simulink library "Multibody_Parts_Lib"  (R2025a)
settings: Solver=VariableStepAuto  StartTime=0.0  StopTime=10.0  RelTol=1e-3
undefined symbols (not defined in the file): b_gear_pd_asy, b_radius_asy, b_visc_frict_asy, bevel_angle_asy, bevel_angle_bf_asy, bevel_angle_fg_asy, f_gear_pd_asy, f_radius_asy, f_visc_frict_asy, g_radius_asy, g_visc_frict_asy, gear_ra_asy, gear_visc_frict_asy, Hand, Left, Local, pinion_pd_asy, screw_lead, worm_lead_angle_asy, worm_rad_asy, worm_visc_frict_asy, X, Y, Z
libraries: sm_lib x143, $bdroot x22, nesl_utility x16
(part 1 of 6)
Description:
  | Simscape Multibody Parts Library v4.0
  | Copyright 2018-2025 The MathWorks, Inc.
settings Model: Creator=smiller  LastModifiedBy=smiller
settings SolverCC: AlgebraicLoopSolver=TrustRegion
settings DataIOCC: ReturnWorkspaceOutputs=off
settings OptimizationCC: ReuseModelBlockBuffer=off
settings DebuggingCC: UnconnectedInputMsg=warning  UnconnectedOutputMsg=warning  UnconnectedLineMsg=warning  PregeneratedLibrarySubsystemCodeDiagnostic=none  ArithmeticOperatorsInVariantConditions=warning
settings ModelReferenceCC: EnableRefExpFcnMdlSchedulingChecks=on
settings SFSimCC: SimUseLocalCustomCode=off  CustomCodeUndefinedFunction=UseInterfaceOnly
settings RTWCC: RTWUseLocalCustomCode=off  GPUComputeCapability=3.5  DLArmComputeVersion=19.05
settings CodeAppCC: StateflowObjectComments=on

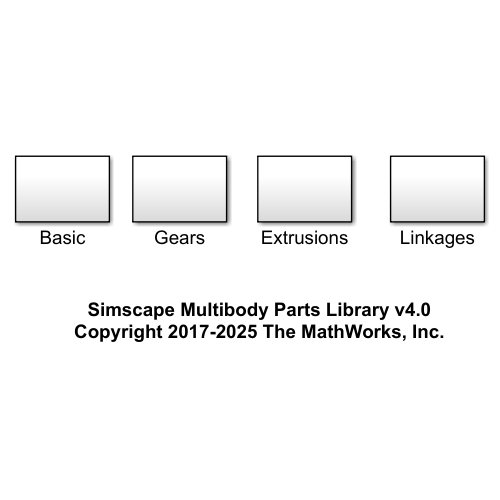
[thumbnail: Simulink's stored preview of the top-level diagram]
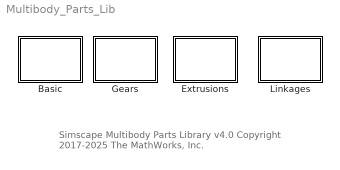
== system Multibody_Parts_Lib ==
  note: Simscape Multibody Parts Library v4.0
      | Copyright 2017-2025 The MathWorks, Inc.
  Basic : Subsystem
  Extrusions : Subsystem
  Gears : Subsystem
  Linkages : Subsystem

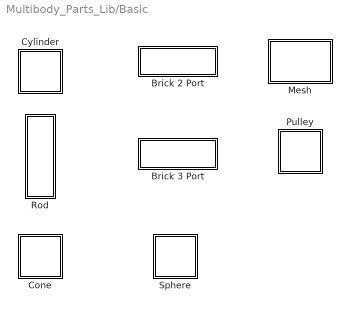
== system Multibody_Parts_Lib/Basic ==
  Brick 2 Port : Subsystem  mask(Brick with 2 Interface Frames){len_xyz=[0.1 0.2 0.3], brick_rho=7000, brick_clr=[0.6 0.6 0.6], brick_opc=1, popup_port1=+X, popup_port2=+X, port1_offset=[0 0 0]}
      mask prompts: len_xyz "Length [X Y Z] (m)"; brick_rho "Density (kg/m^3)"; brick_clr "Color [RGB]"; brick_opc "Opacity (0-1)"; popup_port1 "Port 1 Face"; popup_port2 "Port 2 Face"
      mask help: This block models a brick. The two interface ports can be configured to be at the center of any of the six faces. The orientation of the frames is the same.
      mask init:
      | f=Simulink.FindOptions('FollowLinks',1,'LookUnderMasks','all');
      | p1_h=Simulink.findBlocks(gcb,'Port','1',f);
      | p2_h=Simulink.findBlocks(gcb,'Port','2',f);
      | 
      | switch(popup_port1)
      |     case 1, port1_offset = [ len_xyz(1)/2 0 0]; port1_name = '1X';
      |     case 2, port1_offset = [-len_xyz(1)/2 0 0];  port1_name = '1-X';
      |     case 3, port1_offset = [ 0  len_xyz(2)/2 0];  port1_name = '1Y';
      |     case 4, port1_offset = [ 0 -len_xyz(2)/2 0];  port1_name = '1-Y';
      |     case 5, port1_offset = [ 0  0  len_xyz(3)/2]; port1_name = '1Z';
      |     case 6, port1_offset = [ 0  0 -len_xyz(3)/2]; port1_name = '1-Z';
      | end
      | 
      | switch(popup_port2)
      |     case 1, port2_offset = [ len_xyz(1)/2 0 0]; port2_name = 'X2';
      |     case 2, port2_offset = [-len_xyz(1)/2 0 0];  port2_name = '-X2';
      |     case 3, port2_offset = [ 0  len_xyz(2)/2 0];  port2_name = 'Y2';
      |     case 4, port2_offset = [ 0 -len_xyz(2)/2 0];  port2_name = '-Y2';
      |     case 5, port2_offset = [ 0  0  len_xyz(3)/2]; port2_name = 'Z2';
      |     case 6, port2_offset = [ 0  0 -len_xyz(3)/2]; port2_name = '-Z2';
      | end
      | 
      | set_param(p1_h,'Name',port1_name);
      | set_param(p2_h,'Name',port2_name);
      mask TypeOptions popup_port1: +X | -X | +Y | -Y | +Z | -Z
      mask TypeOptions popup_port2: +X | -X | +Y | -Y | +Z | -Z
      mask Display: image('Brick_2_Port_IMAGE.png')
  Brick 3 Port : Subsystem  mask(Brick with 3 Interface Frames){len_xyz=[0.1 0.2 0.3], brick_rho=7000, brick_clr=[0.6 0.6 0.6], brick_opc=1, popup_port1=+X, popup_port2=+X, popup_port3=+X, port1_offset=[0 0 0]}
      mask prompts: len_xyz "Length [X Y Z] (m)"; brick_rho "Density (kg/m^3)"; brick_clr "Color [RGB]"; brick_opc "Opacity (0-1)"; popup_port1 "Port 1 Face"; popup_port2 "Port 2 Face"; popup_port3 "Port 3 Face"
      mask help: This block models a brick. The three interface ports can be configured to be at the center of any of the six faces. The orientation of the frames is the same.
      mask init:
      | f=Simulink.FindOptions('FollowLinks',1,'LookUnderMasks','all');
      | p1_h=Simulink.findBlocks(gcb,'Port','1',f);
      | p2_h=Simulink.findBlocks(gcb,'Port','2',f);
      | p3_h=Simulink.findBlocks(gcb,'Port','3',f);
      | 
      | switch(popup_port1)
      |     case 1, port1_offset = [ len_xyz(1)/2 0 0]; port1_name = '1X';
      |     case 2, port1_offset = [-len_xyz(1)/2 0 0];  port1_name = '1-X';
      |     case 3, port1_offset = [ 0  len_xyz(2)/2 0];  port1_name = '1Y';
      |     case 4, port1_offset = [ 0 -len_xyz(2)/2 0];  port1_name = '1-Y';
      |     case 5, port1_offset = [ 0  0  len_xyz(3)/2]; port1_name = '1Z';
      |     case 6, port1_offset = [ 0  0 -len_xyz(3)/2]; port1_name = '1-Z';
      | end
      | 
      | switch(popup_port2)
      |     case 1, port2_offset = [ len_xyz(1)/2 0 0]; port2_name = 'X2';
      |     case 2, port2_offset = [-len_xyz(1)/2 0 0];  port2_name = '-X2';
      |     case 3, port2_offset = [ 0  len_xyz(2)/2 0];  port2_name = 'Y2';
      |     case 4, port2_offset = [ 0 -len_xyz(2)/2 0];  port2_name = '-Y2';
      |     case 5, port2_offset = [ 0  0  len_xyz(3)/2]; port2_name = 'Z2';
      |     case 6, port2_offset = [ 0  0 -len_xyz(3)/2]; port2_name = '-Z2';
      | end
      | 
      | switch(popup_port3)
      |     case 1, port3_offset = [ len_xyz(1)/2 0 0]; port3_name = 'X3';
      |     case 2, port3_offset = [-len_xyz(1)/2 0 0];  port3_name = '-X3';
      |     case 3, port3_offset = [ 0  len_xyz(2)/2 0];  port3_name = 'Y3';
      |     case 4, port3_offset = [ 0 -len_xyz(2)/2 0];  port3_name = '-Y3';
      |     case 5, port3_offset = [ 0  0  len_xyz(3)/2]; port3_name = 'Z3';
      |     case 6, port3_offset = [ 0  0 -len_xyz(3)/2]; port3_name = '-Z3';
      | end
      | 
      | set_param(p1_h,'Name',port1_name);
      | set_param(p2_h,'Name',port2_name);
      | set_param(p3_h,'Name',port3_name);
      mask TypeOptions popup_port1: +X | -X | +Y | -Y | +Z | -Z
      mask TypeOptions popup_port2: +X | -X | +Y | -Y | +Z | -Z
      mask TypeOptions popup_port3: +X | -X | +Y | -Y | +Z | -Z
      mask Display: image('Brick_3_Port_IMAGE.png');
  Cone : Subsystem  mask(Conical Frustum){cone_or=37.5e-3, cone_ir=30e-3, cone_h=4e-2, cone_theta=60, cone_angle_range=[-180 180], cone_rho=7000, cone_clr=[0.0 0.4 0.6], cone_opc=1, popup_markings=Two, mark_radius_scale=[1.01 1.01], mark_angle_range=2, mark_color=[1 1 1]}
      mask prompts: cone_or "Outer Radius (m):"; cone_ir "Inner Radius (m):"; cone_h "Height (m):"; cone_theta "Angle (deg):"; cone_angle_range "Sweep Angle (min, max angle (deg))"; cone_rho "Density (kg/m^3):"; cone_clr "Color [RGB]:"; cone_opc "Opacity (0-1)"; popup_markings "Show Markings"; mark_radius_scale "Radius scale factor [rad, h] (~1)"; mark_angle_range "Sweep Angle [0-180] (deg)"; mark_color "Color [RGB]"
      mask help:
      | This block models a conical frustum.
      |
      | The port C corresponds to the frame at one end of the cone whose z-axis points along the cone axis.
      mask init:
      | frcon_xsec = Extr_Data_Frustum_Conical(cone_or, cone_theta, cone_h, cone_ir);
      | mark_xsec = Extr_Data_Frustum_Conical(cone_or*mark_radius_scale(1), cone_theta, cone_h*(1+(mark_radius_scale(2)-1)*2), cone_ir*(2-mark_radius_scale(1)));
      | 
      | mark_xsec(:,2) = mark_xsec(:,2)-cone_h*(mark_radius_scale(2)-1);
      | 
      | mark_1_opc = 0;
      | mark_2_opc = 0;
      | 
      | if(popup_markings == 2)
      |     mark_1_opc = 1;
      | elseif(popup_markings == 3)
      |     mark_1_opc = 1;
      |     mark_2_opc = 1;
      | end
      mask TypeOptions popup_markings: None | One | Two
      mask Callback popup_markings:
      | maskObj = Simulink.Mask.get(gcb);
      | mkc_h = maskObj.getDialogControl('container_markings');
      | if strcmp(get_param(gcb,'popup_markings'),'None')
      |     mkc_h.Visible = 'off';
      | else
      |     mkc_h.Visible = 'on';
      | end
      | clear maskObj mkc_h
      mask DialogControl Control2 Prompt: Plot Profile
      mask DialogControl Control2 Callback:
      | v = get_param(gcb,'MaskWSVariables');
      | getMaskValue = containers.Map({v.Name}',{v.Value}');
      | evalin('base',...
      |     sprintf('Extr_Data_Frustum_Conical(%s,%s,%s,%s,''%s'');',...
      |     num2str(getMaskValue('cone_or')),...
      |     num2str(getMaskValue('cone_theta')),...
      |     num2str(getMaskValue('cone_h')),...
      |     num2str(getMaskValue('cone_ir')),'plot'));
      mask Display: image('Cone_IMAGE.png');
  Cylinder : Subsystem  mask(Cylinder with Hole){cyl_ra=37.5e-3, cyl_th=9e-3, cyl_hr=5e-3, cyl_rho=7000, cyl_clr=[0.6 0.6 0.6], cyl_opc=1, popup_markings=Two, mark_radius_range=[0.7 0.9], mark_angle_range=60, mark_color=[1 1 1]}
      mask prompts: cyl_ra "Radius (m):"; cyl_th "Length (m):"; cyl_hr "Hole Radius (m):"; cyl_rho "Density (kg/m^3):"; cyl_clr "Color [RGB]:"; cyl_opc "Opacity (0-1):"; popup_markings "Show Markings"; mark_radius_range "Radial Range [min max] (0-1)"; mark_angle_range "Sweep Angle [0-180] (deg)"; mark_color "Color [RGB]"
      mask help:
      | This block models a cylinder with a hole for the shaft.
      |
      | The port C corresponds to the frame at the center of the cylinder.
      mask init:
      | cyl_xsec = [cyl_hr -cyl_th/2;
      |              cyl_ra -cyl_th/2;
      |              cyl_ra cyl_th/2;
      |              cyl_hr cyl_th/2];
      | mark_xsec =  [
      |     cyl_ra*max(mark_radius_range) cyl_th/1.9; 
      |     cyl_ra*min(mark_radius_range) cyl_th/1.9; 
      |     cyl_ra*min(mark_radius_range) -cyl_th/1.9; 
      |     cyl_ra*max(mark_radius_range) -cyl_th/1.9];
      | 
      | mark_1_opc = 0;
      | mark_2_opc = 0;
      | 
      | if(popup_markings == 2)
      |     mark_1_opc = 1;
      | elseif(popup_markings == 3)
      |     mark_1_opc = 1;
      |     mark_2_opc = 1;
      | end
      mask TypeOptions popup_markings: None | One | Two
      mask Callback popup_markings:
      | maskObj = Simulink.Mask.get(gcb);
      | mkc_h = maskObj.getDialogControl('container_markings');
      | if strcmp(get_param(gcb,'popup_markings'),'None')
      |     mkc_h.Visible = 'off';
      | else
      |     mkc_h.Visible = 'on';
      | end
      | clear maskObj mkc_h
      mask Display: image('Cylinder_IMAGE.png');
  Mesh : Subsystem  mask(Rectangular Mesh){mesh_lenx=0.6, mesh_leny=0.4, mesh_hx=0.18, mesh_hy=0.18, mesh_numhx=3, mesh_numhy=2, mesh_thickness=0.02, mesh_rho=7000, mesh_color=[0 0.4 0.6], mesh_opc=1}
      mask prompts: mesh_thickness "Thickness (m)"; mesh_rho "Density (kg/m^3)"; mesh_color "Color [RGB]"; mesh_opc "Opacity (0-1)"
      mask help: Rectangular mesh. Define outer dimensions, dimensions of holes, and thickness. R port is at the CG. Thickness defines the distance of the F frame from the B frame along the z-axis.
      mask init:
      | mesh_xsec = Extr_Data_Mesh(mesh_lenx, mesh_leny, mesh_numhx, mesh_numhy, mesh_hx, mesh_hy);
      mask DialogControl Control12 Prompt: Plot Profile
      mask DialogControl Control12 Callback:
      | v = get_param(gcb,'MaskWSVariables');
      | getMaskValue = containers.Map({v.Name}',{v.Value}');
      | evalin('base',...
      |     sprintf('Extr_Data_Mesh(%s,%s,%s,%s,%s,%s,''%s'');',...
      |     num2str(getMaskValue('mesh_lenx')),...
      |     num2str(getMaskValue('mesh_leny')),...
      |     num2str(getMaskValue('mesh_numhx')),...
      |     num2str(getMaskValue('mesh_numhy')),...
      |     num2str(getMaskValue('mesh_hx')),...
      |     num2str(getMaskValue('mesh_hy')),'plot'));
      mask DialogControl Control7 Prompt: X
      mask DialogControl Control8 Prompt: Y
      mask DialogControl Control9 Prompt: Mesh Length (m)
      mask DialogControl Control11 Prompt: Hole Length (m)
      mask DialogControl Control10 Prompt: Number of Holes
      mask Display: image('Mesh_IMAGE.png');
  Pulley : Subsystem  mask(Pulley with Hole){pulley_rad=0.02, pulley_d_grv=0.005, pulley_a_grv=45, pulley_th=0.01, pulley_radh=0.005, pulley_rho=7000, pulley_clr=[0.6 0.6 0.6], pulley_opc=1, pulley_zori=No, popup_markings=Two, mark_radius_range=[0.7 0.9], mark_angle_range=60, mark_color=[1 1 1]}
      mask prompts: pulley_rad "Radius for Cable (m):"; pulley_d_grv "Groove Depth (m):"; pulley_a_grv "Groove Angle (deg):"; pulley_th "Pulley Thickness (m):"; pulley_radh "Hole Radius (m):"; pulley_rho "Density (kg/m^3):"; pulley_clr "Color [RGB]:"; pulley_opc "Opacity (0-1)"; pulley_zori "Flip Z Axis"; popup_markings "Show Markings"; mark_radius_range "Radial Range [min max] (0-1)"; mark_angle_range "Sweep Angle [0-180] (deg)"; mark_color "Color [RGB]"
      mask help:
      | This block models a pulley with a groove for a cable and a hole for the shaft.
      |
      | The port C corresponds to the frame at the center of the pulley.
      mask init:
      | pulley_xsec = Extr_Data_Pulley(...
      |     pulley_rad, pulley_d_grv, pulley_radh,...
      |     pulley_a_grv, pulley_th);
      | 
      | mark_xsec =  [
      |     pulley_rad*max(mark_radius_range) pulley_th/1.9; 
      |     pulley_rad*min(mark_radius_range) pulley_th/1.9; 
      |     pulley_rad*min(mark_radius_range) -pulley_th/1.9; 
      |     pulley_rad*max(mark_radius_range) -pulley_th/1.9];
      | 
      | mark_1_opc = 0;
      | mark_2_opc = 0;
      | 
      | if(pulley_zori == 1)
      |  set_param([gcb '/Transform Swap Z'],'RotationMethod','None'),
      | elseif(pulley_zori == 2)
      |  set_param([gcb '/Transform Swap Z'],'RotationMethod','StandardAxis','RotationStandardAxis','+X'),
      | elseif(pulley_zori == 3)
      |  set_param([gcb '/Transform Swap Z'],'RotationMethod','StandardAxis','RotationStandardAxis','+Y'),
      | end    
      | 
      | if(popup_markings == 2)
      |     mark_1_opc = 1;
      | elseif(popup_markings == 3)
      |     mark_1_opc = 1;
      |     mark_2_opc = 1;
      | end
      mask TypeOptions pulley_zori: No | Yes, about X | Yes, about Y
      mask TypeOptions popup_markings: None | One | Two
      mask Callback popup_markings:
      | maskObj = Simulink.Mask.get(gcb);
      | mkc_h = maskObj.getDialogControl('container_markings');
      | if strcmp(get_param(gcb,'popup_markings'),'None')
      |     mkc_h.Visible = 'off';
      | else
      |     mkc_h.Visible = 'on';
      | end
      | clear maskObj mkc_h
      mask DialogControl Control2 Prompt: Plot Profile
      mask DialogControl Control2 Callback:
      | v = get_param(gcb,'MaskWSVariables');
      | getMaskValue = containers.Map({v.Name}',{v.Value}');
      | evalin('base',...
      |     sprintf('Extr_Data_Pulley(%s,%s,%s,%s,%s,''%s'');',...
      |     num2str(getMaskValue('pulley_rad')),...
      |     num2str(getMaskValue('pulley_d_grv')),...
      |     num2str(getMaskValue('pulley_radh')),...
      |     num2str(getMaskValue('pulley_a_grv')),...
      |     num2str(getMaskValue('pulley_th')),'plot'));
      mask Display: image('Pulley_IMAGE.png');
  Rod : Subsystem  mask(Rod){rod_rad=0.005, rod_len=0.0125, rod_rho=7000, rod_color=[0.5 0.5 0.5], rod_opc=1, popup_zori=Local +Z, popup_markings=None, mark_radius_range=[0.5 1.01], mark_length_range=1.005, mark_angle_range=30, mark_color=[1 1 1]}
      mask prompts: rod_rad "Radius (m)"; rod_len "Length (m)"; rod_rho "Density (kg/m^3)"; rod_color "Color [RGB]"; rod_opc "Opacity (0-1)"; popup_zori "Relative Position (B to F)"; popup_markings "Show Markings"; mark_radius_range "Radial Range [min max] (0-1.1)"; mark_length_range "Length Range (0-1.1)"; mark_angle_range "Sweep Angle [0-180] (deg)"; mark_color "Color [RGB]"
      mask help:
      | This block models a rod.
      |
      | The two interface ports corresponds to the frames at either end of the rod which are along the z-axis.
      mask init:
      | mark_xsec =  [
      |     rod_rad*max(mark_radius_range) rod_len*mark_length_range/2; 
      |     rod_rad*min(mark_radius_range) rod_len*mark_length_range/2; 
      |     rod_rad*min(mark_radius_range) -rod_len*mark_length_range/2; 
      |     rod_rad*max(mark_radius_range) -rod_len*mark_length_range/2];
      | 
      | mark_1_opc = 0;
      | mark_2_opc = 0;
      | 
      | if(popup_markings == 2)
      |     mark_1_opc = 1;
      | elseif(popup_markings == 3)
      |     mark_1_opc = 1;
      |     mark_2_opc = 1;
      | end
      | 
      | if(popup_zori == 2)
      |     z_ori = -1;
      | else
      |     z_ori = 1;
      | end
      mask TypeOptions popup_zori: Local +Z | Local -Z
      mask TypeOptions popup_markings: None | One | Two
      mask Callback popup_markings:
      | maskObj = Simulink.Mask.get(gcb);
      | mkc_h = maskObj.getDialogControl('container_markings');
      | if strcmp(get_param(gcb,'popup_markings'),'None')
      |     mkc_h.Visible = 'off';
      | else
      |     mkc_h.Visible = 'on';
      | end
      | clear maskObj mkc_h
      mask Display:
      | if(popup_zori == 2)
      |     image('Rod_nZ_IMAGE.png')
      | else
      |     image('Rod_pZ_IMAGE.png')
      | end
  Sphere : Subsystem  Tag=CustomStyle  mask(Sphere){sph_radius=0.01, sph_density=1000, sph_color=[0 0.4 0.6], sph_opacity=1, mark_type=Arcs about axes, arc_width=[40 50], arc_angle=60, ring_width=5, ring_irad=0.95, mark_color_popup=Axes, mark_color=[0.2 0.2 0.2], mark_color_x=[1 0 0];, mark_color_y=[0 1 0];, mark_color_z=[0 0 1];, mark_opacity_x=1, mark_opacity_y=1, mark_opacity_z=1, mark_opacity=1, ring_opacity=0, arc_opacity=0, arc_extr_data=0}
      mask prompts: sph_radius "Radius (m)"; sph_density "Density (kg/m^3)"; sph_color "Color [RGB]"; sph_opacity "Opacity"; mark_type "Marking Type"; arc_width "Arc width (start, end) (deg)"; arc_angle "Sweep angle (deg)"; ring_width "Ring Width (deg)"; ring_irad "Ring Inner Radius (% sphere radius)"; mark_color_popup "Color Scheme"; mark_color "Color [RGB]"; mark_opacity_x "Opacity (0-1): X-Axis"; mark_opacity_y "Y-Axis"; mark_opacity_z "Z-Axis"; mark_opacity "Opacity"; ring_opacity "Ring Opacity"; arc_opacity "Arc Opacity"; arc_extr_data "Arc Extrusion Data (xy)"
      mask help:
      | This block models a sphere.
      |
      | The port C corresponds to the frame at the center of the sphere.
      mask init:
      | curblk = gcb;
      | 
      | if strcmp(get_param(curblk,'mark_color_popup'),'Axes')
      |     mark_color_x = [1.0 0.0 0.0];
      |     mark_color_y = [0.0 1.0 0.0];
      |     mark_color_z = [0.0 0.0 1.0];
      | else
      |     mark_color_x = mark_color;
      |     mark_color_y = mark_color;
      |     mark_color_z = mark_color;
      | end
      | 
      | arc_opacity = 0;
      | ring_opacity = 0;
      | 
      | if strcmp(get_param(curblk,'mark_type'),'Arcs about axes')
      |     arc_opacity = 1;
      | elseif strcmp(get_param(curblk,'mark_type'),'Rings on center planes')
      |     ring_opacity = 1;
      | end
      | 
      | arc_extr_data = sph_radius*1.0001*[cosd(min(arc_width):(max(arc_width)-min(arc_width))/20:max(arc_width)) cosd(-max(arc_width):(max(arc_width)-min(arc_width))/20:-min(arc_width)); sind(min(arc_width):(max(arc_width)-min(arc_width))/20:max(arc_width)) sind(-max(arc_width):(max(arc_width)-min(arc_width))/20:-min(arc_width))]';
      | clear curblk
      mask TypeOptions mark_type: None | Arcs about axes | Rings on center planes
      mask Callback mark_type:
      | maskObj = Simulink.Mask.get(gcb);
      | arw_h = maskObj.getParameter('arc_width');
      | ara_h = maskObj.getParameter('arc_angle');
      | riw_h = maskObj.getParameter('ring_width');
      | rii_h = maskObj.getParameter('ring_irad');
      | mkp_h = maskObj.getParameter('mark_color_popup');
      | mkc_h = maskObj.getParameter('mark_color');
      | opx_h = maskObj.getParameter('mark_opacity_x');
      | opy_h = maskObj.getParameter('mark_opacity_y');
      | opz_h = maskObj.getParameter('mark_opacity_z');
      |     arw_h.Visible = 'off';
      |     ara_h.Visible = 'off';
      |     riw_h.Visible = 'off';
      |     rii_h.Visible = 'off';
      |     mkp_h.Visible = 'off';
      |     mkc_h.Visible = 'off';
      |     opx_h.Visible = 'off';
      |     opy_h.Visible = 'off';
      |     opz_h.Visible = 'off';
      | if strcmp(get_param(gcb,'mark_type'),'Arcs about axes')
      |     arw_h.Visible = 'on';
      |     ara_h.Visible = 'on';
      |     mkp_h.Visible = 'on';
      |     mkc_h.Visible = 'on';
      |     opx_h.Visible = 'on';
      |     opy_h.Visible = 'on';
      |     opz_h.Visible = 'on';
      | elseif strcmp(get_param(gcb,'mark_type'),'Rings on center planes')
      |     riw_h.Visible = 'on';
      |     rii_h.Visible = 'on';
      |     mkp_h.Visible = 'on';
      |     opx_h.Visible = 'on';
      |     opy_h.Visible = 'on';
      |     opz_h.Visible = 'on';
      | end
      | clear maskObj
      mask TypeOptions mark_color_popup: Axes | Custom
      mask Callback mark_color_popup:
      | maskObj = Simulink.Mask.get(gcb);
      | mkc_h = maskObj.getParameter('mark_color');
      | if strcmp(get_param(gcb,'mark_color_popup'),'Custom')
      |  mkc_h.Visible = 'on';
      | else
      |  mkc_h.Visible = 'off';
      | end
      | clear maskObj
      mask DialogControl Container4 Prompt: Sphere
      mask DialogControl Container7 Prompt: Markings
      mask Display: image('Sphere_IMAGE.png')

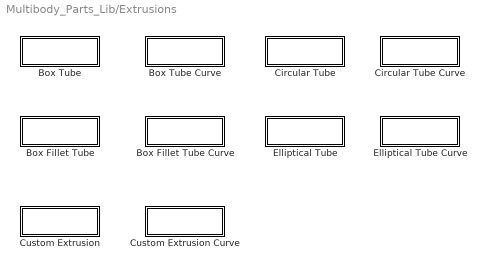
== system Multibody_Parts_Lib/Extrusions ==
  Box Fillet Tube : Subsystem  mask(Box Tube with Filleted Corners){box_ox=0.02, box_ix=0.01, box_oy=0.028, box_iy=0.018, rad_o=0.005, rad_i=0.002, box_len=0.5, box_rho=7000, box_color=[0 0.4 0.6], box_opc=1}
      mask prompts: box_len "Length (m)"; box_rho "Density (kg/m^3)"; box_color "Color [RGB]"; box_opc "Opacity (0-1)"
      mask help: Box tube with rounded corners. Define outer dimensions, inner dimensions, and length. Length defines the distance of the +X frame from the X frame along the x-axis.
      mask init:
      | box_xsec = Extr_Data_BoxFillet(box_ox, box_oy, rad_o, box_ix, box_iy, rad_i);
      mask DialogControl Control12 Prompt: Plot Profile
      mask DialogControl Control12 Callback:
      | v = get_param(gcb,'MaskWSVariables');
      | getMaskValue = containers.Map({v.Name}',{v.Value}');
      | evalin('base',...
      |     sprintf('Extr_Data_BoxFillet(%s,%s,%s,%s,%s,%s,''%s'');',...
      |     num2str(getMaskValue('box_ox')),...
      |     num2str(getMaskValue('box_oy')),...
      |     num2str(getMaskValue('rad_o')),...
      |     num2str(getMaskValue('box_ix')),...
      |     num2str(getMaskValue('box_iy')),...
      |     num2str(getMaskValue('rad_i')),'plot'));
      mask DialogControl Control3 Prompt: Outer
      mask DialogControl Control4 Prompt: Inner
      mask DialogControl Control5 Prompt: Width (m)
      mask DialogControl Control6 Prompt: Height (m)
      mask DialogControl Control7 Prompt: Fillet (m)
      mask Display: image('Box_Fillet_Tube_IMAGE.png');
  Box Fillet Tube Curve : Subsystem  mask(Box Tube with Curve){box_ox=0.02, box_ix=0.01, box_oy=0.028, box_iy=0.018, rad_o=0.005, rad_i=0.002, arc_rad=0.5, arc_angle=-60, popup_arcdir=Y, box_rho=7000, box_color=[0 0.4 0.6], box_opc=1}
      mask prompts: arc_rad "Arc Radius (m)"; arc_angle "Arc Angle (deg)"; popup_arcdir "About"; box_rho "Density (kg/m^3)"; box_color "Color [RGB]"; box_opc "Opacity (0-1)"
      mask help: Box tube. Define outer dimensions, inner dimensions, and length. Length defines the distance of the F frame from the B frame along the z-axis.
      mask init:
      | box_xsec = Extr_Data_BoxFillet(box_ox, box_oy, rad_o, box_ix, box_iy, rad_i);
      | 
      | % Transform extrusion data based on curve axis and direction
      | if (arc_angle<0)
      |     if(strcmpi(get_param(gcb,'popup_arcdir'),'y'))
      |         box_xsec_d = flipud(box_xsec.*[1 -1]);
      |         Bzrot = -90-arc_angle/2;
      |         Fzrot = -90+arc_angle/2;
      |     elseif(strcmpi(get_param(gcb,'popup_arcdir'),'z'))
      |         box_xsec_d = fliplr(box_xsec).*[1 -1];
      |         Bzrot = 90+arc_angle/2;
      |         Fzrot = -90+arc_angle/2;
      |     end
      | else
      |     if(strcmpi(get_param(gcb,'popup_arcdir'),'y'))
      |         box_xsec_d = flipud(box_xsec.*[-1 1]);
      |     elseif(strcmpi(get_param(gcb,'popup_arcdir'),'z'))
      |         box_xsec_d = -flipud(fliplr(box_xsec));
      |     end
      |     Bzrot = -90+arc_angle/2;
      |     Fzrot = 90+arc_angle/2;
      | end
      | 
      | % Add offset for arc radius
      | box_xsec_d = box_xsec_d + [arc_rad 0];
      | 
      | % Adjust Base and Follower transforms based on curve axis
      | if(strcmpi(get_param(gcb,'popup_arcdir'),'y'))
      |     set_param([gcb '/Transform B'],'TranslationStandardAxis','-Z');
      |     set_param([gcb '/Transform B'],'RotationSequenceAngles','[-90*sign(arc_angle) Bzrot 0]');
      |     set_param([gcb '/Transform F'],'RotationSequenceAngles','[90*sign(arc_angle) Fzrot 0]');
      |     set_param([gcb '/Transform F'],'TranslationThetaOffset','arc_angle/2*sign(arc_angle)')
      | else
      |     set_param([gcb '/Transform B'],'TranslationStandardAxis','+Y');
      |     set_param([gcb '/Transform B'],'RotationSequenceAngles','[0 Bzrot 0]');
      |     set_param([gcb '/Transform F'],'RotationSequenceAngles','[0 0 Fzrot]');
      |     set_param([gcb '/Transform F'],'TranslationThetaOffset','arc_angle/2');
      | end
      mask TypeOptions popup_arcdir: Y | Z
      mask DialogControl Control12 Prompt: Plot Profile
      mask DialogControl Control12 Callback:
      | v = get_param(gcb,'MaskWSVariables');
      | getMaskValue = containers.Map({v.Name}',{v.Value}');
      | evalin('base',...
      |     sprintf('Extr_Data_BoxFillet(%s,%s,%s,%s,%s,%s,''%s'');',...
      |     num2str(getMaskValue('box_ox')),...
      |     num2str(getMaskValue('box_oy')),...
      |     num2str(getMaskValue('rad_o')),...
      |     num2str(getMaskValue('box_ix')),...
      |     num2str(getMaskValue('box_iy')),...
      |     num2str(getMaskValue('rad_i')),'plot'));
      mask DialogControl Control3 Prompt: Outer
      mask DialogControl Control4 Prompt: Inner
      mask DialogControl Control5 Prompt: Width (m)
      mask DialogControl Control6 Prompt: Height (m)
      mask DialogControl Control7 Prompt: Fillet (m)
      mask Display: image('Box_Fillet_Tube_Curve_IMAGE.png')
  Box Tube : Subsystem  mask(Box Tube){box_ox=0.02, box_ix=0.01, box_oy=0.028, box_iy=0.018, box_len=0.5, box_rho=7000, box_color=[0 0.4 0.6], box_opc=1}
      mask prompts: box_len "Length (m)"; box_rho "Density (kg/m^3)"; box_color "Color [RGB]"; box_opc "Opacity (0-1)"
      mask help: Box tube. Define outer dimensions, inner dimensions, and length. Length defines the distance of the +X frame from the X frame along the x-axis.
      mask init:
      | box_xsec = Extr_Data_Box(box_ox, box_ix, box_oy, box_iy);
      mask DialogControl Control12 Prompt: Plot Profile
      mask DialogControl Control12 Callback:
      | v = get_param(gcb,'MaskWSVariables');
      | getMaskValue = containers.Map({v.Name}',{v.Value}');
      | evalin('base',...
      |     sprintf('Extr_Data_Box(%s,%s,%s,%s,''%s'');',...
      |     num2str(getMaskValue('box_ox')),...
      |     num2str(getMaskValue('box_ix')),...
      |     num2str(getMaskValue('box_oy')),...
      |     num2str(getMaskValue('box_iy')),'plot'));
      mask DialogControl Control3 Prompt: Outer
      mask DialogControl Control4 Prompt: Inner
      mask DialogControl Control5 Prompt: Width (m)
      mask DialogControl Control6 Prompt: Height (m)
      mask Display: image('Box_Tube_IMAGE.png');
  Box Tube Curve : Subsystem  mask(Box Tube with Curve){box_ox=0.02, box_ix=0.01, box_oy=0.028, box_iy=0.018, arc_rad=0.5, arc_angle=-60, popup_arcdir=Y, box_rho=7000, box_color=[0 0.4 0.6], box_opc=1}
      mask prompts: arc_rad "Arc Radius (m)"; arc_angle "Arc Angle (deg)"; popup_arcdir "About"; box_rho "Density (kg/m^3)"; box_color "Color [RGB]"; box_opc "Opacity (0-1)"
      mask help: Box tube. Define outer dimensions, inner dimensions, and length. Length defines the distance of the F frame from the B frame along the z-axis.
      mask init:
      | box_xsec = Extr_Data_Box(box_ox, box_ix, box_oy, box_iy);
      | 
      | % Transform extrusion data based on curve axis and direction
      | if (arc_angle<0)
      |     if(strcmpi(get_param(gcb,'popup_arcdir'),'y'))
      |         box_xsec_d = flipud(box_xsec.*[1 -1]);
      |         Bzrot = -90-arc_angle/2;
      |         Fzrot = -90+arc_angle/2;
      |     elseif(strcmpi(get_param(gcb,'popup_arcdir'),'z'))
      |         box_xsec_d = fliplr(box_xsec).*[1 -1];
      |         Bzrot = 90+arc_angle/2;
      |         Fzrot = -90+arc_angle/2;
      |     end
      | else
      |     if(strcmpi(get_param(gcb,'popup_arcdir'),'y'))
      |         box_xsec_d = flipud(box_xsec.*[-1 1]);
      |     elseif(strcmpi(get_param(gcb,'popup_arcdir'),'z'))
      |         box_xsec_d = -flipud(fliplr(box_xsec));
      |     end
      |     Bzrot = -90+arc_angle/2;
      |     Fzrot = 90+arc_angle/2;
      | end
      | 
      | % Add offset for arc radius
      | box_xsec_d = box_xsec_d + [arc_rad 0];
      | 
      | % Adjust Base and Follower transforms based on curve axis
      | if(strcmpi(get_param(gcb,'popup_arcdir'),'y'))
      |     set_param([gcb '/Transform B'],'TranslationStandardAxis','-Z');
      |     set_param([gcb '/Transform B'],'RotationSequenceAngles','[-90*sign(arc_angle) Bzrot 0]');
      |     set_param([gcb '/Transform F'],'RotationSequenceAngles','[90*sign(arc_angle) Fzrot 0]');
      |     set_param([gcb '/Transform F'],'TranslationThetaOffset','arc_angle/2*sign(arc_angle)')
      | else
      |     set_param([gcb '/Transform B'],'TranslationStandardAxis','+Y');
      |     set_param([gcb '/Transform B'],'RotationSequenceAngles','[0 Bzrot 0]');
      |     set_param([gcb '/Transform F'],'RotationSequenceAngles','[0 0 Fzrot]');
      |     set_param([gcb '/Transform F'],'TranslationThetaOffset','arc_angle/2');
      | end
      mask TypeOptions popup_arcdir: Y | Z
      mask DialogControl Control12 Prompt: Plot Profile
      mask DialogControl Control12 Callback:
      | v = get_param(gcb,'MaskWSVariables');
      | getMaskValue = containers.Map({v.Name}',{v.Value}');
      | evalin('base',...
      |     sprintf('Extr_Data_Box(%s,%s,%s,%s,''%s'');',...
      |     num2str(getMaskValue('box_ox')),...
      |     num2str(getMaskValue('box_ix')),...
      |     num2str(getMaskValue('box_oy')),...
      |     num2str(getMaskValue('box_iy')),'plot'));
      mask DialogControl Control3 Prompt: Outer
      mask DialogControl Control4 Prompt: Inner
      mask DialogControl Control5 Prompt: Width (m)
      mask DialogControl Control6 Prompt: Height (m)
      mask Display: image('Box_Tube_Curve_IMAGE.png')
  Circular Tube : Subsystem  mask(Elliptical Tube){circ_radout=0.03, circ_radin=0.02, deg_1=45, deg_2=315, circ_len=0.5, circ_rho=7000, circ_color=[0 0.4 0.6], circ_opc=1}
      mask prompts: deg_1 "Start Angle (deg)"; deg_2 "Finish Angle (deg)"; circ_len "Length (m)"; circ_rho "Density (kg/m^3)"; circ_color "Color [RGB]"; circ_opc "Opacity (0-1)"
      mask help: Elliptical tube. Define outer dimensions, hollowness, length, and start and finish angle. Length defines the distance of the F frame from the B frame along the z-axis.
      mask init:
      | circ_xsec = Extr_Data_Ring(circ_radout, circ_radin, deg_1, deg_2);
      mask DialogControl Control12 Prompt: Plot Profile
      mask DialogControl Control12 Callback:
      | v = get_param(gcb,'MaskWSVariables');
      | getMaskValue = containers.Map({v.Name}',{v.Value}');
      | evalin('base',...
      |     sprintf('Extr_Data_Ring(%s,%s,%s,%s,''%s'');',...
      |     num2str(getMaskValue('circ_radout')),...
      |     num2str(getMaskValue('circ_radin')),...
      |     num2str(getMaskValue('deg_1')),...
      |     num2str(getMaskValue('deg_2')),'plot'));
      mask DialogControl Control3 Prompt: Outer
      mask DialogControl Control4 Prompt: Inner
      mask DialogControl Control5 Prompt: Radius (m)
      mask Display: image('Circular_Tube_IMAGE.png')
  Circular Tube Curve : Subsystem  mask(Curved Circular Tube){circ_radout=0.03, circ_radin=0.02, deg_1=45, deg_2=315, arc_rad=0.5, arc_angle=45, popup_arcdir=Y, circ_rho=7000, circ_color=[0 0.4 0.6], circ_opc=1}
      mask prompts: deg_1 "Start Angle (deg)"; deg_2 "Finish Angle (deg)"; arc_rad "Arc Radius (m)"; arc_angle "Arc Angle (deg)"; popup_arcdir "About (axis)"; circ_rho "Density (kg/m^3)"; circ_color "Color [RGB]"; circ_opc "Opacity (0-1)"
      mask help: Elliptical tube. Define outer dimensions, hollowness, length, and start and finish angle. Length defines the distance of the F frame from the B frame along the z-axis.
      mask init:
      | % Generate default extrusion data
      | circ_xsec = Extr_Data_Ring(circ_radout, circ_radin, deg_1, deg_2);
      | 
      | % Transform extrusion data based on curve axis and direction
      | if (arc_angle<0)
      |     if(strcmpi(get_param(gcb,'popup_arcdir'),'y'))
      |         circ_xsec_d = flipud(circ_xsec.*[1 -1]);
      |         Bzrot = -90-arc_angle/2;
      |         Fzrot = -90+arc_angle/2;
      |     elseif(strcmpi(get_param(gcb,'popup_arcdir'),'z'))
      |         circ_xsec_d = fliplr(circ_xsec).*[1 -1];
      |         Bzrot = 90+arc_angle/2;
      |         Fzrot = -90+arc_angle/2;
      |     end
      | else
      |     if(strcmpi(get_param(gcb,'popup_arcdir'),'y'))
      |         circ_xsec_d = flipud(circ_xsec.*[-1 1]);
      |     elseif(strcmpi(get_param(gcb,'popup_arcdir'),'z'))
      |         circ_xsec_d = -flipud(fliplr(circ_xsec));
      |     end
      |     Bzrot = -90+arc_angle/2;
      |     Fzrot = 90+arc_angle/2;
      | end
      | 
      | % Add offset for arc radius
      | circ_xsec_d = circ_xsec_d + [arc_rad 0];
      | 
      | % Adjust Base and Follower transforms based on curve axis
      | if(strcmpi(get_param(gcb,'popup_arcdir'),'y'))
      |     set_param([gcb '/Transform B'],'TranslationStandardAxis','-Z');
      |     set_param([gcb '/Transform B'],'RotationSequenceAngles','[-90*sign(arc_angle) Bzrot 0]');
      |     set_param([gcb '/Transform F'],'RotationSequenceAngles','[90*sign(arc_angle) Fzrot 0]');
      |     set_param([gcb '/Transform F'],'TranslationThetaOffset','arc_angle/2*sign(arc_angle)')
      | else
      |     set_param([gcb '/Transform B'],'TranslationStandardAxis','+Y');
      |     set_param([gcb '/Transform B'],'RotationSequenceAngles','[0 Bzrot 0]');
      |     set_param([gcb '/Transform F'],'RotationSequenceAngles','[0 0 Fzrot]');
      |     set_param([gcb '/Transform F'],'TranslationThetaOffset','arc_angle/2');
      | end
      mask TypeOptions popup_arcdir: Y | Z
      mask DialogControl Control12 Prompt: Plot Profile
      mask DialogControl Control12 Callback:
      | v = get_param(gcb,'MaskWSVariables');
      | getMaskValue = containers.Map({v.Name}',{v.Value}');
      | evalin('base',...
      |     sprintf('Extr_Data_Ring(%s,%s,%s,%s,''%s'');',...
      |     num2str(getMaskValue('circ_radout')),...
      |     num2str(getMaskValue('circ_radin')),...
      |     num2str(getMaskValue('deg_1')),...
      |     num2str(getMaskValue('deg_2')),'plot'));
      mask DialogControl Control3 Prompt: Outer
      mask DialogControl Control4 Prompt: Inner
      mask DialogControl Control5 Prompt: Radius (m)
      mask Display: image('Circular_Tube_Curve_IMAGE.png')
  Custom Extrusion : Subsystem  mask(Box Tube){extr_xsec=[-1 1;-1 -1;1 -1;0.5 -0.5;-0.5 -0.5;-0.5 0.5]*2e-2, extr_len=0.5, extr_rho=7000, extr_color=[0 0.4 0.6], extr_opc=1}
      mask prompts: extr_xsec "Extrusion Data [x y] (m)"; extr_len "Length (m)"; extr_rho "Density (kg/m^3)"; extr_color "Color [RGB]"; extr_opc "Opacity (0-1)"
      mask help: Box tube. Define outer dimensions, inner dimensions, and length. Length defines the distance of the +X frame from the X frame along the x-axis.
      mask DialogControl Control12 Prompt: Plot Profile
      mask DialogControl Control12 Callback:
      | v = get_param(gcb,'MaskWSVariables');
      | getMaskValue = containers.Map({v.Name}',{v.Value}');
      | blk_xydata = getMaskValue('extr_xsec');
      | assignin('base','temp_cust_extr_xy_data',blk_xydata);
      | 
      | evalin('base',...
      |     sprintf('Extr_Data_Custom(temp_cust_extr_xy_data);clear temp_cust_extr_xy_data'));
      mask Display: image('Custom_Extrusion_IMAGE.png');
  Custom Extrusion Curve : Subsystem  mask(Box Tube with Curve){extr_xsec=[-1 1;-1 -1;1 -1;0.5 -0.5;-0.5 -0.5;-0.5 0.5]*2e-2, arc_rad=1.25, arc_angle=-60, popup_arcdir=Y, extr_rho=7000, extr_color=[0 0.4 0.6], extr_opc=1}
      mask prompts: extr_xsec "Extrusion Data [x y] (m)"; arc_rad "Arc Radius (m)"; arc_angle "Arc Angle (deg)"; popup_arcdir "About"; extr_rho "Density (kg/m^3)"; extr_color "Color [RGB]"; extr_opc "Opacity (0-1)"
      mask help: Box tube. Define outer dimensions, inner dimensions, and length. Length defines the distance of the F frame from the B frame along the z-axis.
      mask init:
      | % Transform extrusion data based on curve axis and direction
      | if (arc_angle<0)
      |     if(strcmpi(get_param(gcb,'popup_arcdir'),'y'))
      |         extr_xsec_d = flipud(extr_xsec.*[1 -1]);
      |         Bzrot = -90-arc_angle/2;
      |         Fzrot = -90+arc_angle/2;
      |     elseif(strcmpi(get_param(gcb,'popup_arcdir'),'z'))
      |         extr_xsec_d = fliplr(extr_xsec).*[1 -1];
      |         Bzrot = 90+arc_angle/2;
      |         Fzrot = -90+arc_angle/2;
      |     end
      | else
      |     if(strcmpi(get_param(gcb,'popup_arcdir'),'y'))
      |         extr_xsec_d = flipud(extr_xsec.*[-1 1]);
      |     elseif(strcmpi(get_param(gcb,'popup_arcdir'),'z'))
      |         extr_xsec_d = -flipud(fliplr(extr_xsec));
      |     end
      |     Bzrot = -90+arc_angle/2;
      |     Fzrot = 90+arc_angle/2;
      | end
      | 
      | % Add offset for arc radius
      | extr_xsec_d = extr_xsec_d + [arc_rad 0];
      | 
      | % Adjust Base and Follower transforms based on curve axis
      | if(strcmpi(get_param(gcb,'popup_arcdir'),'y'))
      |     set_param([gcb '/Transform B'],'TranslationStandardAxis','-Z');
      |     set_param([gcb '/Transform B'],'RotationSequenceAngles','[-90*sign(arc_angle) Bzrot 0]');
      |     set_param([gcb '/Transform F'],'RotationSequenceAngles','[90*sign(arc_angle) Fzrot 0]');
      |     set_param([gcb '/Transform F'],'TranslationThetaOffset','arc_angle/2*sign(arc_angle)')
      | else
      |     set_param([gcb '/Transform B'],'TranslationStandardAxis','+Y');
      |     set_param([gcb '/Transform B'],'RotationSequenceAngles','[0 Bzrot 0]');
      |     set_param([gcb '/Transform F'],'RotationSequenceAngles','[0 0 Fzrot]');
      |     set_param([gcb '/Transform F'],'TranslationThetaOffset','arc_angle/2');
      | end
      mask TypeOptions popup_arcdir: Y | Z
      mask DialogControl Control12 Prompt: Plot Profile
      mask DialogControl Control12 Callback:
      | v = get_param(gcb,'MaskWSVariables');
      | getMaskValue = containers.Map({v.Name}',{v.Value}');
      | blk_xydata = getMaskValue('extr_xsec');
      | assignin('base','temp_cust_extr_xy_data',blk_xydata);
      | 
      | evalin('base',...
      |     sprintf('Extr_Data_Custom(temp_cust_extr_xy_data);clear temp_cust_extr_xy_data'));
      mask Display: image('Custom_Extrusion_Curve_IMAGE.png')
  Elliptical Tube : Subsystem  mask(Elliptical Tube){rad_a=0.02, rad_b=0.03, deg_1=10, deg_2=350, ctr=0, ell_len=0.5, ell_rho=7000, ell_color=[0 0.4 0.6], ell_opc=1}
      mask prompts: deg_1 "Start Angle (deg)"; deg_2 "Finish Angle (deg)"; ctr "Center (0-1)"; ell_len "Length (m)"; ell_rho "Density (kg/m^3)"; ell_color "Color [RGB]"; ell_opc "Opacity (0-1)"
      mask help: Elliptical tube. Define outer dimensions, hollowness, length, and start and finish angle. Length defines the distance of the F frame from the B frame along the z-axis.
      mask init:
      | ell_xsec = Extr_Data_Ellipse(rad_a, rad_b, deg_1, deg_2, ctr);
      mask DialogControl Control12 Prompt: Plot Profile
      mask DialogControl Control12 Callback:
      | v = get_param(gcb,'MaskWSVariables');
      | getMaskValue = containers.Map({v.Name}',{v.Value}');evalin('base',...
      |     sprintf('Extr_Data_Ellipse(%s,%s,%s,%s,%s,''%s'');',...
      |     num2str(getMaskValue('rad_a')),...
      |     num2str(getMaskValue('rad_b')),...
      |     num2str(getMaskValue('deg_1')),...
      |     num2str(getMaskValue('deg_2')),...
      |     num2str(getMaskValue('ctr')),'plot'));
      mask DialogControl Control3 Prompt: X-Axis
      mask DialogControl Control4 Prompt: Y-Axis
      mask DialogControl Control5 Prompt: Radius (m)
      mask Display: image('Elliptical_Tube_IMAGE.png')
  Elliptical Tube Curve : Subsystem  mask(Elliptical Tube){rad_a=0.02, rad_b=0.03, deg_1=10, deg_2=350, ctr=0, arc_rad=0.5, arc_angle=45, popup_arcdir=Y, ell_rho=7000, ell_color=[0 0.4 0.6], ell_opc=1}
      mask prompts: deg_1 "Start Angle (deg)"; deg_2 "Finish Angle (deg)"; ctr "Center (0-1)"; arc_rad "Arc Radius (m)"; arc_angle "Arc Angle (deg)"; popup_arcdir "About (axis)"; ell_rho "Density (kg/m^3)"; ell_color "Color [RGB]"; ell_opc "Opacity (0-1)"
      mask help: Elliptical tube. Define outer dimensions, hollowness, length, and start and finish angle. Length defines the distance of the F frame from the B frame along the z-axis.
      mask init:
      | ell_xsec = Extr_Data_Ellipse(rad_a, rad_b, deg_1, deg_2, ctr);
      | 
      | % Transform extrusion data based on curve axis and direction
      | if (arc_angle<0)
      |     if(strcmpi(get_param(gcb,'popup_arcdir'),'y'))
      |         ell_xsec_d = flipud(ell_xsec.*[1 -1]);
      |         Bzrot = -90-arc_angle/2;
      |         Fzrot = -90+arc_angle/2;
      |     elseif(strcmpi(get_param(gcb,'popup_arcdir'),'z'))
      |         ell_xsec_d = fliplr(ell_xsec).*[1 -1];
      |         Bzrot = 90+arc_angle/2;
      |         Fzrot = -90+arc_angle/2;
      |     end
      | else
      |     if(strcmpi(get_param(gcb,'popup_arcdir'),'y'))
      |         ell_xsec_d = flipud(ell_xsec.*[-1 1]);
      |     elseif(strcmpi(get_param(gcb,'popup_arcdir'),'z'))
      |         ell_xsec_d = -flipud(fliplr(ell_xsec));
      |     end
      |     Bzrot = -90+arc_angle/2;
      |     Fzrot = 90+arc_angle/2;
      | end
      | 
      | % Add offset for arc radius
      | ell_xsec_d = ell_xsec_d + [arc_rad 0];
      | 
      | % Adjust Base and Follower transforms based on curve axis
      | if(strcmpi(get_param(gcb,'popup_arcdir'),'y'))
      |     set_param([gcb '/Transform B'],'TranslationStandardAxis','-Z');
      |     set_param([gcb '/Transform B'],'RotationSequenceAngles','[-90*sign(arc_angle) Bzrot 0]');
      |     set_param([gcb '/Transform F'],'RotationSequenceAngles','[90*sign(arc_angle) Fzrot 0]');
      |     set_param([gcb '/Transform F'],'TranslationThetaOffset','arc_angle/2*sign(arc_angle)')
      | else
      |     set_param([gcb '/Transform B'],'TranslationStandardAxis','+Y');
      |     set_param([gcb '/Transform B'],'RotationSequenceAngles','[0 Bzrot 0]');
      |     set_param([gcb '/Transform F'],'RotationSequenceAngles','[0 0 Fzrot]');
      |     set_param([gcb '/Transform F'],'TranslationThetaOffset','arc_angle/2');
      | end
      mask TypeOptions popup_arcdir: Y | Z
      mask DialogControl Control12 Prompt: Plot Profile
      mask DialogControl Control12 Callback:
      | v = get_param(gcb,'MaskWSVariables');
      | getMaskValue = containers.Map({v.Name}',{v.Value}');evalin('base',...
      |     sprintf('Extr_Data_Ellipse(%s,%s,%s,%s,%s,''%s'');',...
      |     num2str(getMaskValue('rad_a')),...
      |     num2str(getMaskValue('rad_b')),...
      |     num2str(getMaskValue('deg_1')),...
      |     num2str(getMaskValue('deg_2')),...
      |     num2str(getMaskValue('ctr')),'plot'));
      mask DialogControl Control3 Prompt: X-Axis
      mask DialogControl Control4 Prompt: Y-Axis
      mask DialogControl Control5 Prompt: Radius (m)
      mask Display: image('Elliptical_Tube_Curve_IMAGE.png')
